simulink model "InsulinPumpModelV7_ParFor"  (R2022b)
settings: Solver=ode23t  StartTime=0.0  StopTime=12  MaxStep=0.001  RelTol=1e-5  EnableMultiTasking=on
undefined symbols (not defined in the file): const_Occl_Pct, DeliveryType, DiscIntNeverNeededParam, MagB, PauseTime, reserv_str, StrokeTimeB
libraries: fl_lib x71, nesl_utility x35, sldvlib x14, sh_lib x9, fl_ps_legacy_lib x8, sdl_lib x7, ee_lib x1, simulink_extras x1, simulink x1, slpidlib x1
(part 2 of 2)

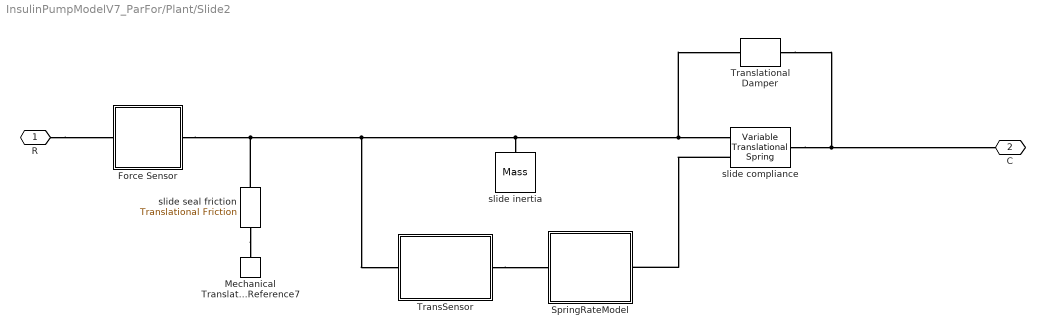
== system InsulinPumpModelV7_ParFor/Plant/Slide2 ==
  Force Sensor : Subsystem
  Mechanical Translational Reference7 : fl_lib/Mechanical/Translational Elements/Mechanical Translational Reference
  SpringRateModel : Subsystem  mask{E=reserv_str.Slide.EMod, A=reserv_str.Slide.CrosA, InitL=reserv_str.Slide.InitL}
      mask prompts: E "Young's Modulus (Pa)"; A "Cross-sectional Area (m^2)"; InitL "Initial Length (m)"
  TransSensor : Subsystem
  Translational Damper : sdl_lib/Couplings & Drives/Springs & Dampers/Translational Damper  D=10000 N/(m/s)  enable_faults=0  b_fault=1e6 N/(m/s)  temporal_fault=0  fault_time=5 s  shock_fault=0  acceleration_limit=100 m/s^2  shock_limit=1  report_fault=(1)-1  thermal_port=simscape.enum.thermaleffects.omit  thermal_mass=50 kJ/K  temperature_specify=off  temperature_priority=High  temperature=300 K  temperature_nominal_specify=off  temperature_nominal_unit=K  temperature_nominal_value=1
  slide compliance : sdl_lib/Couplings & Drives/Springs & Dampers/Variable Translational Spring  Kmin=reserv_str.Slide.MinSprRate N/m  x_specify=on  x_priority=High  x=reserv_str.Slide.InitDeform mm  x_nominal_specify=off  x_nominal_unit=m  x_nominal_value=1
      settings: InternalSimscapePortConfiguration="{\"Bottom\":[],\"Left\":[{\"id\":\"K\",\"label\":\"K\",\"type\":\"input\"},{\"id\":\"R\",\"label\":\"R\",\"type\":\"foundation.mechanical.translational.translational\"}],\"Right\":[{\"id\":\"C\",\"label\":\"C\",\"type\":\"foundation.mechanical.translational.translational\"}],\"Top\":[]}"
  slide inertia : fl_lib/Mechanical/Translational Elements/Mass  mass=reserv_str.Slide.Mass kg  num_ports=foundation.enum.numPorts2.one  v_specify=on  v_priority=High  v=0 m/s  v_nominal_specify=off  v_nominal_unit=m/s  v_nominal_value=1  f_specify=off  f_priority=High  f=0 N  f_nominal_specify=off  f_nominal_unit=N  f_nominal_value=1
  slide seal friction : fl_lib/Mechanical/Translational Elements/Translational Friction  brkwy_frc=reserv_str.Slide.Brkaway N  brkwy_vel=exp(-( (reserv_str.Slide.LinVelThresh) * 1 * (reserv_str.Slide.TransApproxCoeff) * 1 + 1/2) ) * ( (reserv_str.Slide.LinVelThresh) * 1 / 2 + 1 / ( (reserv_str.Slide.TransApproxCoeff) * 1) ) m/s  Col_frc=reserv_str.Slide.Coulomb N  visc_coef=reserv_str.Slide.ViscFric N/(m/s)  v_specify=off  v_priority=High  v=0 m/s  v_nominal_specify=off  v_nominal_unit=m/s  v_nominal_value=1  f_specify=off  f_priority=High  f=0 N  f_nominal_specify=off  f_nominal_unit=N  f_nominal_value=1
      settings: InternalSimscapePortConfiguration="{\"Bottom\":[],\"Left\":[{\"id\":\"R\",\"label\":\"R\",\"type\":\"foundation.mechanical.translational.translational\"}],\"Right\":[{\"id\":\"C\",\"label\":\"C\",\"type\":\"foundation.mechanical.translational.translational\"}],\"Top\":[]}"
  R : PMIOPort  Side=Left
  C : PMIOPort  Port=2  Side=Right
  connections:
  R/RConn1 -- Force Sensor/LConn1
  slide seal friction/RConn1 -- Mechanical Translational Reference7/LConn1
  TransSensor/RConn1 -- SpringRateModel/LConn1
  slide compliance/LConn1 -- SpringRateModel/RConn1
  Translational Damper/RConn1 -- C/RConn1 -- slide compliance/RConn1
  slide inertia/LConn1 -- slide compliance/LConn2 -- Translational Damper/LConn1 -- TransSensor/LConn1 -- slide seal friction/LConn1 -- Force Sensor/RConn1

== system InsulinPumpModelV7_ParFor/Plant/Slide3 ==
  Force Sensor : Subsystem
  Mechanical Translational Reference7 : fl_lib/Mechanical/Translational Elements/Mechanical Translational Reference
  SpringRateModel : Subsystem  mask{E=reserv_str.Slide.EMod, A=reserv_str.Slide.CrosA, InitL=reserv_str.Slide.InitL}
      mask prompts: E "Young's Modulus (Pa)"; A "Cross-sectional Area (m^2)"; InitL "Initial Length (m)"
  TransSensor : Subsystem
  Translational Damper : sdl_lib/Couplings & Drives/Springs & Dampers/Translational Damper  D=1 N/(m/s)  enable_faults=0  b_fault=1e6 N/(m/s)  temporal_fault=0  fault_time=5 s  shock_fault=0  acceleration_limit=100 m/s^2  shock_limit=1  report_fault=(1)-1  thermal_port=simscape.enum.thermaleffects.omit  thermal_mass=50 kJ/K  temperature_specify=off  temperature_priority=High  temperature=300 K  temperature_nominal_specify=off  temperature_nominal_unit=K  temperature_nominal_value=1
  slide compliance : sdl_lib/Couplings & Drives/Springs & Dampers/Variable Translational Spring  Kmin=reserv_str.Slide.MinSprRate N/m  x_specify=on  x_priority=High  x=reserv_str.Slide.InitDeform mm  x_nominal_specify=off  x_nominal_unit=m  x_nominal_value=1
      settings: InternalSimscapePortConfiguration="{\"Bottom\":[],\"Left\":[{\"id\":\"K\",\"label\":\"K\",\"type\":\"input\"},{\"id\":\"R\",\"label\":\"R\",\"type\":\"foundation.mechanical.translational.translational\"}],\"Right\":[{\"id\":\"C\",\"label\":\"C\",\"type\":\"foundation.mechanical.translational.translational\"}],\"Top\":[]}"
  slide inertia : fl_lib/Mechanical/Translational Elements/Mass  mass=reserv_str.Slide.Mass kg  num_ports=foundation.enum.numPorts2.one  v_specify=on  v_priority=High  v=0 m/s  v_nominal_specify=off  v_nominal_unit=m/s  v_nominal_value=1  f_specify=off  f_priority=High  f=0 N  f_nominal_specify=off  f_nominal_unit=N  f_nominal_value=1
  slide seal friction : fl_lib/Mechanical/Translational Elements/Translational Friction  brkwy_frc=reserv_str.Slide.Brkaway N  brkwy_vel=exp(-( (reserv_str.Slide.LinVelThresh) * 1 * (reserv_str.Slide.TransApproxCoeff) * 1 + 1/2) ) * ( (reserv_str.Slide.LinVelThresh) * 1 / 2 + 1 / ( (reserv_str.Slide.TransApproxCoeff) * 1) ) m/s  Col_frc=reserv_str.Slide.Coulomb N  visc_coef=reserv_str.Slide.ViscFric N/(m/s)  v_specify=off  v_priority=High  v=0 m/s  v_nominal_specify=off  v_nominal_unit=m/s  v_nominal_value=1  f_specify=off  f_priority=High  f=0 N  f_nominal_specify=off  f_nominal_unit=N  f_nominal_value=1
      settings: InternalSimscapePortConfiguration="{\"Bottom\":[],\"Left\":[{\"id\":\"R\",\"label\":\"R\",\"type\":\"foundation.mechanical.translational.translational\"}],\"Right\":[{\"id\":\"C\",\"label\":\"C\",\"type\":\"foundation.mechanical.translational.translational\"}],\"Top\":[]}"
  R : PMIOPort  Side=Left
  C : PMIOPort  Port=2  Side=Right
  connections:
  R/RConn1 -- Force Sensor/LConn1
  slide seal friction/RConn1 -- Mechanical Translational Reference7/LConn1
  TransSensor/RConn1 -- SpringRateModel/LConn1
  slide compliance/LConn1 -- SpringRateModel/RConn1
  Translational Damper/RConn1 -- C/RConn1 -- slide compliance/RConn1
  slide seal friction/LConn1 -- Translational Damper/LConn1 -- slide compliance/LConn2 -- slide inertia/LConn1 -- TransSensor/LConn1 -- Force Sensor/RConn1

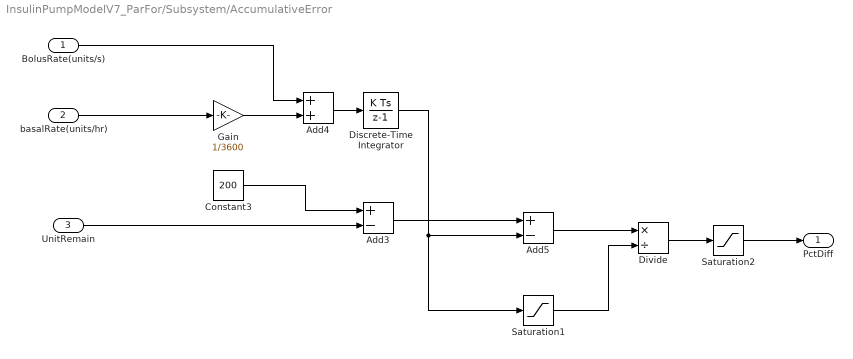
== system InsulinPumpModelV7_ParFor/Subsystem/AccumulativeError ==
  BolusRate(units/s) : Inport
  basalRate(units/hr) : Inport  Port=2
  UnitRemain : Inport  Port=3
  Add3 : Sum  Inputs=+-
  Add4 : Sum
  Add5 : Sum  Inputs=+-
  Constant3 : Constant  Value=200
  Discrete-Time Integrator : DiscreteIntegrator  SampleTime=-1  ICPrevOutput=DiscIntNeverNeededParam  ICPrevScaledInput=DiscIntNeverNeededParam
  Divide : Product  Inputs=*/
  Gain : Gain  Gain=1/3600
  Saturation1 : Saturate  UpperLimit=200  LowerLimit=0.000001
  Saturation2 : Saturate  UpperLimit=1  LowerLimit=-1
  PctDiff : Outport
  wires:
  Divide/1 -> Saturation2/1
  Saturation1/1 -> Divide/2
  UnitRemain/1 -> Add3/2
  basalRate(units/hr)/1 -> Gain/1
  BolusRate(units/s)/1 -> Add4/1
  Add4/1 -> Discrete-Time Integrator/1
  Discrete-Time Integrator/1 -> Add5/2, Saturation1/1
  Add3/1 -> Add5/1
  Constant3/1 -> Add3/1
  Saturation2/1 -> PctDiff/1
  Gain/1 -> Add4/2
  Add5/1 -> Divide/1

== system InsulinPumpModelV7_ParFor/Subsystem/Disp2Unit ==
  Piston_P : Inport  OutMin=-30  OutMax=0
  Add2 : Sum  Inputs=+-
  Add3 : Sum
  Constant : Constant  Value=reserv_str.Resvor.Vol  OutDataTypeStr=single
  Constant1 : Constant  Value=reserv_str.Resvor.Len  OutDataTypeStr=single
  Gain : Gain  Gain=reserv_str.Resvor.Area
  Gain1 : Gain  Gain=1/15
  Scope2 : Scope
  NumU : Outport  OutMin=0  OutMax=201
  wires:
  Constant/1 -> Add2/1
  Constant1/1 -> Add3/2
  Gain/1 -> Add2/2
  Add2/1 -> Gain1/1
  Gain1/1 -> NumU/1
  Add3/1 -> Gain/1, Scope2/1
  Piston_P/1 -> Add3/1

== system InsulinPumpModelV7_ParFor/Subsystem/SpeedController ==
  RefASpd : Inport  OutMin=-6000  OutMax=6000
  ASpd : Inport  Port=2  OutMin=-6000  OutMax=6000
  Add1 : Sum
  Discrete Transfer Fcn2 : DiscreteTransferFcn  Numerator=[0.367879441171442,0.264241117657115]  Denominator=[1,-0.367879441171442]  SampleTime=0.001
  FeedbackController : Subsystem
  Rate Limiter : RateLimiter  RisingSlewLimit=10  FallingSlewLimit=-10  SampleTimeMode=inherited
  Reference_motor_speed_limit : Saturate  UpperLimit=5200  LowerLimit=-5200
  SteadyStateLookup : Lookup_n-D  NumberOfTableDimensions=1  BreakpointsForDimension1=[0 0.136 0.170 0.205 1.08 2.58 8.02 12.8 33.8 828.2 1535.4 2171.5 2526 3000 3827.2 4246 4775.6 4991.1 5209.4]  Table=[0 0.25 0.3 0.35 0.355 0.36 0.38 0.4 0.5 1 1.5 2 2.3 2.72 3.5 3.9 4.4 4.6 4.8]  ExtrapMethod=Clip  InternalRulePriority=Speed  RndMeth=Simplest
  Volt : Outport  OutMin=-10  OutMax=10
  wires:
  RefASpd/1 -> Reference_motor_speed_limit/1
  SteadyStateLookup/1 -> Add1/1
  Discrete Transfer Fcn2/1 -> FeedbackController/1(RefASpd), SteadyStateLookup/1
  Add1/1 -> Rate Limiter/1
  Rate Limiter/1 -> Volt/1
  Reference_motor_speed_limit/1 -> Discrete Transfer Fcn2/1
  FeedbackController/1(Volt) -> Add1/2
  ASpd/1 -> FeedbackController/2(ASpd)

== system InsulinPumpModelV7_ParFor/Subsystem/Units_Conversion ==
  StokeMag : Inport  OutMin=0  OutMax=15
  BasalRate : Inport  Port=2  OutMin=0  OutMax=2
  Add2 : Sum
  BasalMap2Spd : Subsystem
  BolusMap2Spd : Subsystem
  RefASpd : Outport  OutMin=-6000  OutMax=6000
  wires:
  BasalMap2Spd/1(rev/min) -> Add2/2
  BolusMap2Spd/1(rev/min) -> Add2/1
  StokeMag/1 -> BolusMap2Spd/1(unit/s)
  BasalRate/1 -> BasalMap2Spd/1(unit/hr)
  Add2/1 -> RefASpd/1

== system InsulinPumpModelV7_ParFor/Plant/DC Motor Drive/AngSensor ==
  Ideal Rotational Motion Sensor : fl_lib/Mechanical/Mechanical Sensors/Ideal Rotational Motion Sensor  reference=foundation.enum.MeasurementReference.difference  acceleration_port=false  velocity_port=true  position_port=true  wrap_angle=false  offset=0 rad
  Mechanical Rotational Reference1 : fl_lib/Mechanical/Rotational Elements/Mechanical Rotational Reference
  PS-Simulink Converter1 : nesl_utility/PS-Simulink Converter  PhysicalDomain=network_engine_domain  SubClassName=ps_output  LeftPortType=input  RightPortType=output  PseudoPeriodic=off  Frequencies=[]  VectorFormat=1-D array  Unit=rad  AffineConversion=off
  PS-Simulink Converter9 : nesl_utility/PS-Simulink Converter  PhysicalDomain=network_engine_domain  SubClassName=ps_output  LeftPortType=input  RightPortType=output  PseudoPeriodic=off  Frequencies=[]  VectorFormat=1-D array  Unit=rpm  AffineConversion=off
  Terminator1 : Terminator
  R : PMIOPort  Side=Left
  ASpd : Outport
  wires:
  PS-Simulink Converter1/1 -> Terminator1/1  "DCMotor_APos"
  PS-Simulink Converter9/1 -> ASpd/1  "DCMotor_ASpd"
  connections:
  Mechanical Rotational Reference1/LConn1 -- Ideal Rotational Motion Sensor/RConn1
  Ideal Rotational Motion Sensor/RConn2 -- PS-Simulink Converter9/LConn1
  Ideal Rotational Motion Sensor/RConn3 -- PS-Simulink Converter1/LConn1
  R/RConn1 -- Ideal Rotational Motion Sensor/LConn1

== system InsulinPumpModelV7_ParFor/Plant/DC Motor Drive/CurrSensor ==
  Current Sensor1 : fl_lib/Electrical/Electrical Sensors/Current Sensor
  PS-Simulink Converter11 : nesl_utility/PS-Simulink Converter  PhysicalDomain=network_engine_domain  SubClassName=ps_output  LeftPortType=input  RightPortType=output  PseudoPeriodic=off  Frequencies=[]  VectorFormat=1-D array  Unit=A  AffineConversion=off
  Terminator : Terminator
  + : PMIOPort  Side=Left
  - : PMIOPort  Port=2  Side=Right
  wires:
  PS-Simulink Converter11/1 -> Terminator/1
  connections:
  Current Sensor1/RConn2 -- -/RConn1
  Current Sensor1/LConn1 -- +/RConn1
  Current Sensor1/RConn1 -- PS-Simulink Converter11/LConn1

== system InsulinPumpModelV7_ParFor/Plant/DC Motor Drive/TrqSensor ==
  Ideal Torque Sensor1 : fl_lib/Mechanical/Mechanical Sensors/Ideal Torque Sensor
  PS-Simulink Converter10 : nesl_utility/PS-Simulink Converter  PhysicalDomain=network_engine_domain  SubClassName=ps_output  LeftPortType=input  RightPortType=output  PseudoPeriodic=off  Frequencies=[]  VectorFormat=1-D array  Unit=N*m  AffineConversion=off
  Terminator : Terminator
  C : PMIOPort  Side=Right
  R : PMIOPort  Port=2  Side=Left
  wires:
  PS-Simulink Converter10/1 -> Terminator/1  "DCMotor_Torque"
  connections:
  Ideal Torque Sensor1/RConn1 -- C/RConn1
  Ideal Torque Sensor1/RConn2 -- PS-Simulink Converter10/LConn1
  Ideal Torque Sensor1/LConn1 -- R/RConn1

== system InsulinPumpModelV7_ParFor/Plant/DeliveryLine/FlowSensor#0 ==
  Hydraulic Flow Rate Sensor : fl_lib/Hydraulic/Hydraulic Sensors/Hydraulic Flow Rate Sensor
  PS-Simulink Converter : nesl_utility/PS-Simulink Converter  PhysicalDomain=network_engine_domain  SubClassName=ps_output  LeftPortType=input  RightPortType=output  PseudoPeriodic=off  Frequencies=[]  VectorFormat=1-D array  Unit=mm^3/min  AffineConversion=off
  Saturation : Saturate  UpperLimit=inf  LowerLimit=0
  Scope : Scope
  A : PMIOPort  Side=Left
  B : PMIOPort  Port=2  Side=Right
  wires:
  PS-Simulink Converter/1 -> Saturation/1
  Saturation/1 -> Scope/1
  connections:
  Hydraulic Flow Rate Sensor/RConn1 -- PS-Simulink Converter/LConn1
  Hydraulic Flow Rate Sensor/RConn2 -- B/RConn1
  A/RConn1 -- Hydraulic Flow Rate Sensor/LConn1

== system InsulinPumpModelV7_ParFor/Plant/DeliveryLine/FlowSensor#1 ==
  Hydraulic Flow Rate Sensor : fl_lib/Hydraulic/Hydraulic Sensors/Hydraulic Flow Rate Sensor
  PS-Simulink Converter : nesl_utility/PS-Simulink Converter  PhysicalDomain=network_engine_domain  SubClassName=ps_output  LeftPortType=input  RightPortType=output  PseudoPeriodic=off  Frequencies=[]  VectorFormat=1-D array  Unit=mm^3/min  AffineConversion=off
  Saturation : Saturate  Commented=through  UpperLimit=5000  LowerLimit=0
  Scope : Scope
  A : PMIOPort  Side=Left
  B : PMIOPort  Port=2  Side=Right
  wires:
  PS-Simulink Converter/1 -> Saturation/1
  Saturation/1 -> Scope/1
  connections:
  A/RConn1 -- Hydraulic Flow Rate Sensor/LConn1
  Hydraulic Flow Rate Sensor/RConn2 -- B/RConn1
  Hydraulic Flow Rate Sensor/RConn1 -- PS-Simulink Converter/LConn1

== system InsulinPumpModelV7_ParFor/Plant/DeliveryLine/P Sensor ==
  Hydraulic Pressure Sensor : fl_lib/Hydraulic/Hydraulic Sensors/Hydraulic Pressure Sensor
  Hydraulic Reference : fl_lib/Hydraulic/Hydraulic Elements/Hydraulic Reference
  PS-Simulink Converter : nesl_utility/PS-Simulink Converter  PhysicalDomain=network_engine_domain  SubClassName=ps_output  LeftPortType=input  RightPortType=output  PseudoPeriodic=off  Frequencies=[]  VectorFormat=1-D array  Unit=1  AffineConversion=off
  A : PMIOPort  Side=Left
  P : Outport
  wires:
  PS-Simulink Converter/1 -> P/1  "Press2"
  connections:
  Hydraulic Pressure Sensor/RConn1 -- Hydraulic Reference/LConn1
  Hydraulic Pressure Sensor/RConn2 -- PS-Simulink Converter/LConn1
  A/RConn1 -- Hydraulic Pressure Sensor/LConn1

== system InsulinPumpModelV7_ParFor/Plant/Drive System/AngSensor ==
  Ideal Rotational Motion Sensor : fl_lib/Mechanical/Mechanical Sensors/Ideal Rotational Motion Sensor  reference=foundation.enum.MeasurementReference.difference  acceleration_port=false  velocity_port=true  position_port=true  wrap_angle=false  offset=0 rad
  Mechanical Rotational Reference1 : fl_lib/Mechanical/Rotational Elements/Mechanical Rotational Reference
  PS-Simulink Converter1 : nesl_utility/PS-Simulink Converter  PhysicalDomain=network_engine_domain  SubClassName=ps_output  LeftPortType=input  RightPortType=output  PseudoPeriodic=off  Frequencies=[]  VectorFormat=1-D array  Unit=rad  AffineConversion=off
  PS-Simulink Converter9 : nesl_utility/PS-Simulink Converter  PhysicalDomain=network_engine_domain  SubClassName=ps_output  LeftPortType=input  RightPortType=output  PseudoPeriodic=off  Frequencies=[]  VectorFormat=1-D array  Unit=rpm  AffineConversion=off
  Scope : Scope
  Scope1 : Scope
  Terminator : Terminator
  Terminator1 : Terminator
  Conn1 : PMIOPort  Side=Left
  wires:
  PS-Simulink Converter1/1 -> Scope1/1, Terminator1/1  "Inertia_APos"
  PS-Simulink Converter9/1 -> Scope/1, Terminator/1  "Inertia_ASpd"
  connections:
  Mechanical Rotational Reference1/LConn1 -- Ideal Rotational Motion Sensor/RConn1
  Ideal Rotational Motion Sensor/RConn2 -- PS-Simulink Converter9/LConn1
  Ideal Rotational Motion Sensor/RConn3 -- PS-Simulink Converter1/LConn1
  Conn1/RConn1 -- Ideal Rotational Motion Sensor/LConn1

== system InsulinPumpModelV7_ParFor/Plant/Reservoir1/P Sensor ==
  Hydraulic Pressure Sensor : fl_lib/Hydraulic/Hydraulic Sensors/Hydraulic Pressure Sensor
  Hydraulic Reference : fl_lib/Hydraulic/Hydraulic Elements/Hydraulic Reference
  PS-Simulink Converter : nesl_utility/PS-Simulink Converter  PhysicalDomain=network_engine_domain  SubClassName=ps_output  LeftPortType=input  RightPortType=output  PseudoPeriodic=off  Frequencies=[]  VectorFormat=1-D array  Unit=1  AffineConversion=off
  Scope1 : Scope
  A : PMIOPort  Side=Left
  wires:
  PS-Simulink Converter/1 -> Scope1/1  "Press1"
  connections:
  Hydraulic Pressure Sensor/RConn1 -- Hydraulic Reference/LConn1
  Hydraulic Pressure Sensor/RConn2 -- PS-Simulink Converter/LConn1
  A/RConn1 -- Hydraulic Pressure Sensor/LConn1

== system InsulinPumpModelV7_ParFor/Plant/Reservoir1/TransSensor ==
  Ideal Translational Motion Sensor : fl_lib/Mechanical/Mechanical Sensors/Ideal Translational Motion Sensor  reference=foundation.enum.MeasurementReference.difference  acceleration_port=false  velocity_port=true  position_port=true  offset=0 m
  Mechanical Translational Reference1 : fl_lib/Mechanical/Translational Elements/Mechanical Translational Reference
  PS-Simulink Converter3 : nesl_utility/PS-Simulink Converter  PhysicalDomain=network_engine_domain  SubClassName=ps_output  LeftPortType=input  RightPortType=output  PseudoPeriodic=off  Frequencies=[]  VectorFormat=1-D array  Unit=mm/min  AffineConversion=off
  PS-Simulink Converter4 : nesl_utility/PS-Simulink Converter  PhysicalDomain=network_engine_domain  SubClassName=ps_output  LeftPortType=input  RightPortType=output  PseudoPeriodic=off  Frequencies=[]  VectorFormat=1-D array  Unit=mm  AffineConversion=off
  Scope : Scope
  Scope1 : Scope
  Terminator : Terminator
  Terminator1 : Terminator
  Conn1 : PMIOPort  Side=Left
  P : PMIOPort  Port=2  Side=Right
  wires:
  PS-Simulink Converter4/1 -> Scope1/1, Terminator1/1  "Piston_P"
  PS-Simulink Converter3/1 -> Scope/1, Terminator/1  "Piston_V"
  connections:
  Conn1/RConn1 -- Ideal Translational Motion Sensor/LConn1
  Ideal Translational Motion Sensor/RConn3 -- P/RConn1 -- PS-Simulink Converter4/LConn1
  PS-Simulink Converter3/LConn1 -- Ideal Translational Motion Sensor/RConn2
  Mechanical Translational Reference1/LConn1 -- Ideal Translational Motion Sensor/RConn1

== system InsulinPumpModelV7_ParFor/Plant/Reservoir2/P Sensor ==
  Hydraulic Pressure Sensor : fl_lib/Hydraulic/Hydraulic Sensors/Hydraulic Pressure Sensor
  Hydraulic Reference : fl_lib/Hydraulic/Hydraulic Elements/Hydraulic Reference
  PS-Simulink Converter : nesl_utility/PS-Simulink Converter  PhysicalDomain=network_engine_domain  SubClassName=ps_output  LeftPortType=input  RightPortType=output  PseudoPeriodic=off  Frequencies=[]  VectorFormat=1-D array  Unit=1  AffineConversion=off
  Scope1 : Scope
  A : PMIOPort  Side=Left
  wires:
  PS-Simulink Converter/1 -> Scope1/1  "Press1"
  connections:
  A/RConn1 -- Hydraulic Pressure Sensor/LConn1
  Hydraulic Pressure Sensor/RConn2 -- PS-Simulink Converter/LConn1
  Hydraulic Pressure Sensor/RConn1 -- Hydraulic Reference/LConn1

== system InsulinPumpModelV7_ParFor/Plant/Reservoir2/TransSensor ==
  Ideal Translational Motion Sensor : fl_lib/Mechanical/Mechanical Sensors/Ideal Translational Motion Sensor  reference=foundation.enum.MeasurementReference.difference  acceleration_port=false  velocity_port=true  position_port=true  offset=0 m
  Mechanical Translational Reference1 : fl_lib/Mechanical/Translational Elements/Mechanical Translational Reference
  PS-Simulink Converter3 : nesl_utility/PS-Simulink Converter  PhysicalDomain=network_engine_domain  SubClassName=ps_output  LeftPortType=input  RightPortType=output  PseudoPeriodic=off  Frequencies=[]  VectorFormat=1-D array  Unit=mm/min  AffineConversion=off
  PS-Simulink Converter4 : nesl_utility/PS-Simulink Converter  PhysicalDomain=network_engine_domain  SubClassName=ps_output  LeftPortType=input  RightPortType=output  PseudoPeriodic=off  Frequencies=[]  VectorFormat=1-D array  Unit=mm  AffineConversion=off
  Scope : Scope
  Scope1 : Scope
  Terminator : Terminator
  Terminator1 : Terminator
  Conn1 : PMIOPort  Side=Left
  P : PMIOPort  Port=2  Side=Right
  wires:
  PS-Simulink Converter3/1 -> Terminator/1, Scope/1  "Piston_V"
  PS-Simulink Converter4/1 -> Terminator1/1, Scope1/1  "Piston_P"
  connections:
  Mechanical Translational Reference1/LConn1 -- Ideal Translational Motion Sensor/RConn1
  PS-Simulink Converter3/LConn1 -- Ideal Translational Motion Sensor/RConn2
  PS-Simulink Converter4/LConn1 -- P/RConn1 -- Ideal Translational Motion Sensor/RConn3
  Conn1/RConn1 -- Ideal Translational Motion Sensor/LConn1

== system InsulinPumpModelV7_ParFor/Plant/Reservoir3/P Sensor ==
  Hydraulic Pressure Sensor : fl_lib/Hydraulic/Hydraulic Sensors/Hydraulic Pressure Sensor
  Hydraulic Reference : fl_lib/Hydraulic/Hydraulic Elements/Hydraulic Reference
  PS-Simulink Converter : nesl_utility/PS-Simulink Converter  PhysicalDomain=network_engine_domain  SubClassName=ps_output  LeftPortType=input  RightPortType=output  PseudoPeriodic=off  Frequencies=[]  VectorFormat=1-D array  Unit=1  AffineConversion=off
  Scope1 : Scope
  A : PMIOPort  Side=Left
  wires:
  PS-Simulink Converter/1 -> Scope1/1  "Press1"
  connections:
  A/RConn1 -- Hydraulic Pressure Sensor/LConn1
  Hydraulic Pressure Sensor/RConn2 -- PS-Simulink Converter/LConn1
  Hydraulic Pressure Sensor/RConn1 -- Hydraulic Reference/LConn1

== system InsulinPumpModelV7_ParFor/Plant/Reservoir3/TransSensor ==
  Ideal Translational Motion Sensor : fl_lib/Mechanical/Mechanical Sensors/Ideal Translational Motion Sensor  reference=foundation.enum.MeasurementReference.difference  acceleration_port=false  velocity_port=true  position_port=true  offset=0 m
  Mechanical Translational Reference1 : fl_lib/Mechanical/Translational Elements/Mechanical Translational Reference
  PS-Simulink Converter3 : nesl_utility/PS-Simulink Converter  PhysicalDomain=network_engine_domain  SubClassName=ps_output  LeftPortType=input  RightPortType=output  PseudoPeriodic=off  Frequencies=[]  VectorFormat=1-D array  Unit=mm/min  AffineConversion=off
  PS-Simulink Converter4 : nesl_utility/PS-Simulink Converter  PhysicalDomain=network_engine_domain  SubClassName=ps_output  LeftPortType=input  RightPortType=output  PseudoPeriodic=off  Frequencies=[]  VectorFormat=1-D array  Unit=mm  AffineConversion=off
  Scope : Scope
  Scope1 : Scope
  Terminator : Terminator
  Terminator1 : Terminator
  Conn1 : PMIOPort  Side=Left
  P : PMIOPort  Port=2  Side=Right
  wires:
  PS-Simulink Converter3/1 -> Terminator/1, Scope/1  "Piston_V"
  PS-Simulink Converter4/1 -> Terminator1/1, Scope1/1  "Piston_P"
  connections:
  Mechanical Translational Reference1/LConn1 -- Ideal Translational Motion Sensor/RConn1
  PS-Simulink Converter3/LConn1 -- Ideal Translational Motion Sensor/RConn2
  PS-Simulink Converter4/LConn1 -- P/RConn1 -- Ideal Translational Motion Sensor/RConn3
  Conn1/RConn1 -- Ideal Translational Motion Sensor/LConn1

== system InsulinPumpModelV7_ParFor/Plant/Slide1/Force Sensor ==
  Ideal Force Sensor1 : fl_lib/Mechanical/Mechanical Sensors/Ideal Force Sensor
  PS-Simulink Converter15 : nesl_utility/PS-Simulink Converter  PhysicalDomain=network_engine_domain  SubClassName=ps_output  LeftPortType=input  RightPortType=output  PseudoPeriodic=off  Frequencies=[]  VectorFormat=1-D array  Unit=N  AffineConversion=off
  Rate Transition4 : RateTransition  OutPortSampleTime=0.01
  Scope2 : Scope
  Terminator : Terminator
  C : PMIOPort  Side=Right
  R : PMIOPort  Port=2  Side=Left
  wires:
  PS-Simulink Converter15/1 -> Rate Transition4/1, Terminator/1  "Slide_Force"
  Rate Transition4/1 -> Scope2/1
  connections:
  Ideal Force Sensor1/LConn1 -- R/RConn1
  PS-Simulink Converter15/LConn1 -- Ideal Force Sensor1/RConn2
  C/RConn1 -- Ideal Force Sensor1/RConn1

== system InsulinPumpModelV7_ParFor/Plant/Slide2/Force Sensor ==
  Ideal Force Sensor1 : fl_lib/Mechanical/Mechanical Sensors/Ideal Force Sensor
  PS-Simulink Converter15 : nesl_utility/PS-Simulink Converter  PhysicalDomain=network_engine_domain  SubClassName=ps_output  LeftPortType=input  RightPortType=output  PseudoPeriodic=off  Frequencies=[]  VectorFormat=1-D array  Unit=N  AffineConversion=off
  Rate Transition4 : RateTransition  OutPortSampleTime=0.01
  Scope2 : Scope
  Terminator : Terminator
  C : PMIOPort  Side=Right
  R : PMIOPort  Port=2  Side=Left
  wires:
  Rate Transition4/1 -> Scope2/1
  PS-Simulink Converter15/1 -> Terminator/1, Rate Transition4/1  "Slide_Force"
  connections:
  C/RConn1 -- Ideal Force Sensor1/RConn1
  PS-Simulink Converter15/LConn1 -- Ideal Force Sensor1/RConn2
  Ideal Force Sensor1/LConn1 -- R/RConn1

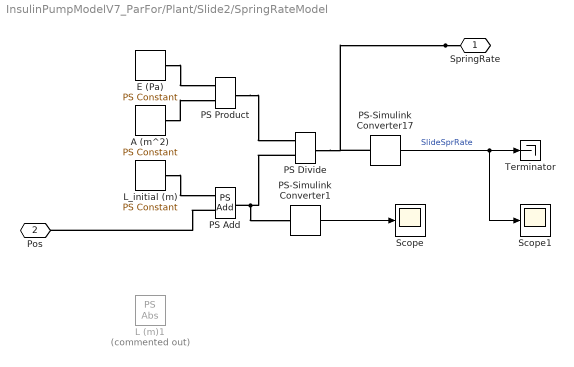
== system InsulinPumpModelV7_ParFor/Plant/Slide2/SpringRateModel ==
  A (m^2) : fl_lib/Physical Signals/Sources/PS Constant  constant=A
  E (Pa) : fl_lib/Physical Signals/Sources/PS Constant  constant=E
  L (m)1 : fl_ps_legacy_lib/Legacy Physical Signals/Nonlinear Operators/PS Abs  Commented=on
      settings: InternalSimscapePortConfiguration="{\"Bottom\":[],\"Left\":[{\"id\":\"I\",\"label\":\"\",\"type\":\"input\"}],\"Right\":[{\"id\":\"O\",\"label\":\"\",\"type\":\"output\"}],\"Top\":[]}"
  L_initial (m) : fl_lib/Physical Signals/Sources/PS Constant  constant=InitL
  PS Add : fl_ps_legacy_lib/Legacy Physical Signals/Functions/PS Add
      settings: InternalSimscapePortConfiguration="{\"Bottom\":[],\"Left\":[{\"id\":\"I1\",\"label\":\"\",\"type\":\"input\"},{\"id\":\"I2\",\"label\":\"\",\"type\":\"input\"}],\"Right\":[{\"id\":\"O\",\"label\":\"\",\"type\":\"output\"}],\"Top\":[]}"
  PS Divide : fl_ps_legacy_lib/Legacy Physical Signals/Functions/PS Divide
      settings: InternalSimscapePortConfiguration="{\"Bottom\":[],\"Left\":[{\"id\":\"I1\",\"label\":\"\",\"type\":\"input\"},{\"id\":\"I2\",\"label\":\"\",\"type\":\"input\"}],\"Right\":[{\"id\":\"O\",\"label\":\"\",\"type\":\"output\"}],\"Top\":[]}"
  PS Product : fl_ps_legacy_lib/Legacy Physical Signals/Functions/PS Product
  PS-Simulink Converter1 : nesl_utility/PS-Simulink Converter  PhysicalDomain=network_engine_domain  SubClassName=ps_output  LeftPortType=input  RightPortType=output  PseudoPeriodic=off  Frequencies=[]  VectorFormat=1-D array  Unit=N/m  AffineConversion=off
  PS-Simulink Converter17 : nesl_utility/PS-Simulink Converter  PhysicalDomain=network_engine_domain  SubClassName=ps_output  LeftPortType=input  RightPortType=output  PseudoPeriodic=off  Frequencies=[]  VectorFormat=1-D array  Unit=N/m  AffineConversion=off
  Scope : Scope
  Scope1 : Scope
  Terminator : Terminator
  SpringRate : PMIOPort  Side=Right
  Pos : PMIOPort  Port=2  Side=Left
  wires:
  PS-Simulink Converter1/1 -> Scope/1
  PS-Simulink Converter17/1 -> Terminator/1, Scope1/1  "SlideSprRate"
  connections:
  PS Add/LConn2 -- Pos/RConn1
  PS Add/RConn1 -- PS-Simulink Converter1/LConn1 -- PS Divide/LConn2
  L_initial (m)/RConn1 -- PS Add/LConn1
  SpringRate/RConn1 -- PS-Simulink Converter17/LConn1 -- PS Divide/RConn1
  PS Product/RConn1 -- PS Divide/LConn1
  A (m^2)/RConn1 -- PS Product/LConn2
  E (Pa)/RConn1 -- PS Product/LConn1

== system InsulinPumpModelV7_ParFor/Plant/Slide2/TransSensor ==
  Ideal Translational Motion Sensor : fl_lib/Mechanical/Mechanical Sensors/Ideal Translational Motion Sensor  reference=foundation.enum.MeasurementReference.difference  acceleration_port=false  velocity_port=true  position_port=true  offset=0 m
  Mechanical Translational Reference1 : fl_lib/Mechanical/Translational Elements/Mechanical Translational Reference
  PS-Simulink Converter3 : nesl_utility/PS-Simulink Converter  PhysicalDomain=network_engine_domain  SubClassName=ps_output  LeftPortType=input  RightPortType=output  PseudoPeriodic=off  Frequencies=[]  VectorFormat=1-D array  Unit=mm/s  AffineConversion=off
  PS-Simulink Converter4 : nesl_utility/PS-Simulink Converter  PhysicalDomain=network_engine_domain  SubClassName=ps_output  LeftPortType=input  RightPortType=output  PseudoPeriodic=off  Frequencies=[]  VectorFormat=1-D array  Unit=mm  AffineConversion=off
  Terminator : Terminator
  Terminator1 : Terminator
  Conn1 : PMIOPort  Side=Left
  P : PMIOPort  Port=2  Side=Right
  wires:
  PS-Simulink Converter3/1 -> Terminator/1  "Slide_V"
  PS-Simulink Converter4/1 -> Terminator1/1  "Slide_P"
  connections:
  Mechanical Translational Reference1/LConn1 -- Ideal Translational Motion Sensor/RConn1
  PS-Simulink Converter3/LConn1 -- Ideal Translational Motion Sensor/RConn2
  PS-Simulink Converter4/LConn1 -- P/RConn1 -- Ideal Translational Motion Sensor/RConn3
  Conn1/RConn1 -- Ideal Translational Motion Sensor/LConn1

== system InsulinPumpModelV7_ParFor/Plant/Slide3/Force Sensor ==
  Ideal Force Sensor1 : fl_lib/Mechanical/Mechanical Sensors/Ideal Force Sensor
  PS-Simulink Converter15 : nesl_utility/PS-Simulink Converter  PhysicalDomain=network_engine_domain  SubClassName=ps_output  LeftPortType=input  RightPortType=output  PseudoPeriodic=off  Frequencies=[]  VectorFormat=1-D array  Unit=N  AffineConversion=off
  Rate Transition4 : RateTransition  OutPortSampleTime=0.01
  Scope2 : Scope
  Terminator : Terminator
  C : PMIOPort  Side=Right
  R : PMIOPort  Port=2  Side=Left
  wires:
  Rate Transition4/1 -> Scope2/1
  PS-Simulink Converter15/1 -> Terminator/1, Rate Transition4/1  "Slide_Force"
  connections:
  C/RConn1 -- Ideal Force Sensor1/RConn1
  PS-Simulink Converter15/LConn1 -- Ideal Force Sensor1/RConn2
  Ideal Force Sensor1/LConn1 -- R/RConn1

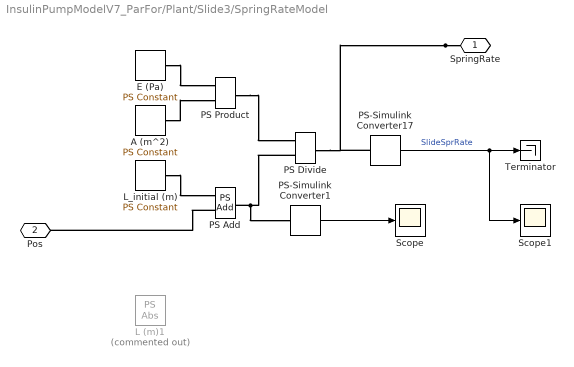
== system InsulinPumpModelV7_ParFor/Plant/Slide3/SpringRateModel ==
  A (m^2) : fl_lib/Physical Signals/Sources/PS Constant  constant=A
  E (Pa) : fl_lib/Physical Signals/Sources/PS Constant  constant=E
  L (m)1 : fl_ps_legacy_lib/Legacy Physical Signals/Nonlinear Operators/PS Abs  Commented=on
      settings: InternalSimscapePortConfiguration="{\"Bottom\":[],\"Left\":[{\"id\":\"I\",\"label\":\"\",\"type\":\"input\"}],\"Right\":[{\"id\":\"O\",\"label\":\"\",\"type\":\"output\"}],\"Top\":[]}"
  L_initial (m) : fl_lib/Physical Signals/Sources/PS Constant  constant=InitL
  PS Add : fl_ps_legacy_lib/Legacy Physical Signals/Functions/PS Add
      settings: InternalSimscapePortConfiguration="{\"Bottom\":[],\"Left\":[{\"id\":\"I1\",\"label\":\"\",\"type\":\"input\"},{\"id\":\"I2\",\"label\":\"\",\"type\":\"input\"}],\"Right\":[{\"id\":\"O\",\"label\":\"\",\"type\":\"output\"}],\"Top\":[]}"
  PS Divide : fl_ps_legacy_lib/Legacy Physical Signals/Functions/PS Divide
      settings: InternalSimscapePortConfiguration="{\"Bottom\":[],\"Left\":[{\"id\":\"I1\",\"label\":\"\",\"type\":\"input\"},{\"id\":\"I2\",\"label\":\"\",\"type\":\"input\"}],\"Right\":[{\"id\":\"O\",\"label\":\"\",\"type\":\"output\"}],\"Top\":[]}"
  PS Product : fl_ps_legacy_lib/Legacy Physical Signals/Functions/PS Product
  PS-Simulink Converter1 : nesl_utility/PS-Simulink Converter  PhysicalDomain=network_engine_domain  SubClassName=ps_output  LeftPortType=input  RightPortType=output  PseudoPeriodic=off  Frequencies=[]  VectorFormat=1-D array  Unit=N/m  AffineConversion=off
  PS-Simulink Converter17 : nesl_utility/PS-Simulink Converter  PhysicalDomain=network_engine_domain  SubClassName=ps_output  LeftPortType=input  RightPortType=output  PseudoPeriodic=off  Frequencies=[]  VectorFormat=1-D array  Unit=N/m  AffineConversion=off
  Scope : Scope
  Scope1 : Scope
  Terminator : Terminator
  SpringRate : PMIOPort  Side=Right
  Pos : PMIOPort  Port=2  Side=Left
  wires:
  PS-Simulink Converter1/1 -> Scope/1
  PS-Simulink Converter17/1 -> Terminator/1, Scope1/1  "SlideSprRate"
  connections:
  PS Add/LConn2 -- Pos/RConn1
  PS Add/RConn1 -- PS-Simulink Converter1/LConn1 -- PS Divide/LConn2
  L_initial (m)/RConn1 -- PS Add/LConn1
  SpringRate/RConn1 -- PS-Simulink Converter17/LConn1 -- PS Divide/RConn1
  PS Product/RConn1 -- PS Divide/LConn1
  A (m^2)/RConn1 -- PS Product/LConn2
  E (Pa)/RConn1 -- PS Product/LConn1

== system InsulinPumpModelV7_ParFor/Plant/Slide3/TransSensor ==
  Ideal Translational Motion Sensor : fl_lib/Mechanical/Mechanical Sensors/Ideal Translational Motion Sensor  reference=foundation.enum.MeasurementReference.difference  acceleration_port=false  velocity_port=true  position_port=true  offset=0 m
  Mechanical Translational Reference1 : fl_lib/Mechanical/Translational Elements/Mechanical Translational Reference
  PS-Simulink Converter3 : nesl_utility/PS-Simulink Converter  PhysicalDomain=network_engine_domain  SubClassName=ps_output  LeftPortType=input  RightPortType=output  PseudoPeriodic=off  Frequencies=[]  VectorFormat=1-D array  Unit=mm/s  AffineConversion=off
  PS-Simulink Converter4 : nesl_utility/PS-Simulink Converter  PhysicalDomain=network_engine_domain  SubClassName=ps_output  LeftPortType=input  RightPortType=output  PseudoPeriodic=off  Frequencies=[]  VectorFormat=1-D array  Unit=mm  AffineConversion=off
  Terminator : Terminator
  Terminator1 : Terminator
  Conn1 : PMIOPort  Side=Left
  P : PMIOPort  Port=2  Side=Right
  wires:
  PS-Simulink Converter3/1 -> Terminator/1  "Slide_V"
  PS-Simulink Converter4/1 -> Terminator1/1  "Slide_P"
  connections:
  Mechanical Translational Reference1/LConn1 -- Ideal Translational Motion Sensor/RConn1
  PS-Simulink Converter3/LConn1 -- Ideal Translational Motion Sensor/RConn2
  PS-Simulink Converter4/LConn1 -- P/RConn1 -- Ideal Translational Motion Sensor/RConn3
  Conn1/RConn1 -- Ideal Translational Motion Sensor/LConn1

== system InsulinPumpModelV7_ParFor/Subsystem/SpeedController/FeedbackController ==
  RefASpd : Inport  OutMin=-6000  OutMax=6000
  ASpd : Inport  Port=2  OutMin=-6000  OutMax=6000
  1-D Lookup Table : Lookup_n-D  NumberOfTableDimensions=1  BreakpointsForDimension1=[0 12.8 33.8 450]  Table=[1 1 1 1]*5e-4  InternalRulePriority=Speed  RndMeth=Simplest
  1-D Lookup Table1 : Lookup_n-D  NumberOfTableDimensions=1  BreakpointsForDimension1=[0 12.8 33.8 450]  Table=[1 1 1 1]*5e-4  InternalRulePriority=Speed  RndMeth=Simplest
  Add : Sum  Inputs=+-
  PID Controller : slpidlib/PID Controller  Controller=PI  Form=Parallel  TimeDomain=Discrete-time  UseExternalTs=off  SampleTime=0.001  IntegratorMethod=Forward Euler  FilterMethod=Forward Euler  ControllerParametersSource=external  P=2e-3  I=2e-3  UseKiTs=off  D=0  N=100  UseFilter=on  TunerSelectOption=Transfer Function Based (PID Tuner App)  InitialConditionSource=internal  InitialConditionForIntegrator=0  InitialConditionForFilter=0  DifferentiatorICPrevScaledInput=0  ExternalReset=none  TrackingMode=off  Kt=1  LimitOutput=off  SatLimitsSource=internal  UpperSaturationLimit=1  LowerSaturationLimit=1  LinearizeAsGain=on  AntiWindupMode=clamping  Kb=1  LimitIntegrator=off  UpperIntegratorSaturationLimit=inf  LowerIntegratorSaturationLimit=-inf  POutMin=[]  POutMax=[]  IOutMin=[]  IOutMax=[]  DOutMin=[]  DOutMax=[]  NOutMin=[]  NOutMax=[]  SumOutMin=[]  SumOutMax=[]  SaturationOutMin=[]  SaturationOutMax=[]  PParamMin=[]  PParamMax=[]  IParamMin=[]  IParamMax=[]  DParamMin=[]  DParamMax=[]  NParamMin=[]  NParamMax=[]  KbParamMin=[]  KbParamMax=[]  KtParamMin=[]  KtParamMax=[]  KbOutMin=[]  KbOutMax=[]  KtOutMin=[]  KtOutMax=[]  IntegratorOutMin=[]  IntegratorOutMax=[]  FilterOutMin=[]  FilterOutMax=[]  SumI1OutMin=[]  SumI1OutMax=[]  SumI2OutMin=[]  SumI2OutMax=[]  SumI3OutMin=[]  SumI3OutMax=[]  SumI4OutMin=[]  SumI4OutMax=[]  SumDOutMin=[]  SumDOutMax=[]  DifferentiatorOutMin=[]  DifferentiatorOutMax=[]  FilterDiffOutCoefMin=[]  FilterDiffOutCoefMax=[]  ReciprocalOutMin=[]  ReciprocalOutMax=[]  SumDenOutMin=[]  SumDenOutMax=[]  SumNumOutMin=[]  SumNumOutMax=[]  DivideOutMin=[]  DivideOutMax=[]  UdiffTsProdOutMin=[]  UdiffTsProdOutMax=[]  NTsProdOutMin=[]  NTsProdOutMax=[]  UintegralTsProdOutMin=[]  UintegralTsProdOutMax=[]  UngainTsProdOutMin=[]  UngainTsProdOutMax=[]  ClampingZeroOutDataTypeStr=Inherit: Inherit via back propagation  ClampingZeroOutMin=[]  ClampingZeroOutMax=[]  FilterDenConstantOutDataTypeStr=Inherit: Inherit via back propagation  FilterDenConstantOutMin=[]  FilterDenConstantOutMax=[]  PCopyOutDataTypeStr=Inherit: Inherit via back propagation  PCopyOutMin=[]  PCopyOutMax=[]  NCopyOutDataTypeStr=Inherit: Inherit via back propagation  NCopyOutMin=[]  NCopyOutMax=[]  IntegratorContinuousStateAttributes=''  IntegratorStateMustResolveToSignalObject=off  IntegratorRTWStateStorageClass=Auto  FilterContinuousStateAttributes=''  FilterStateMustResolveToSignalObject=off  FilterRTWStateStorageClass=Auto  ParallelPVariant=ExternalParameters  IdealPVariant=Disabled  IVariant=ExternalParameters  DVariant=Disabled  IntegratorVariant=Discrete  SatVariant=Disabled  AWVariant=Passthrough  PCopyVariant=Disabled  TRVariant=Disabled  FdbkBlocksVariant=Forward  IdealPFdbkVariant=Disabled  SatFdbkVariant=Disabled  DerivativeFilterVariant=Disabled  NVariant=Disabled  NCopyVariant=Disabled_SignalSpec  FilterICVariant=Disabled  IntegratorICVariant=InternalICs  ExternalResetVariant=Disabled  TRSumVariant=Passthrough  SumFdbkVariant=Disabled  SumVariant=Sum_PI  TsampFilterVariant=InternalTs  TsampNgainVariant=Passthrough  TsampIntegralVariant=Passthrough  ExternalSaturationOutDataTypeStr=Inherit: Same as second input
  Volt : Outport  OutMin=-10  OutMax=10
  wires:
  ASpd/1 -> Add/2
  Add/1 -> 1-D Lookup Table1/1, 1-D Lookup Table/1, PID Controller/1
  PID Controller/1 -> Volt/1
  1-D Lookup Table/1 -> PID Controller/2
  1-D Lookup Table1/1 -> PID Controller/3
  RefASpd/1 -> Add/1

== system InsulinPumpModelV7_ParFor/Subsystem/Units_Conversion/BasalMap2Spd ==
  unit/hr : Inport
  1/CrossArea_Output(mm/min) : Gain  Gain=1/reserv_str.Resvor.Area
  Gain : Gain  Gain=1/60
  Gain3 : Gain  Gain=15
  Gear_Input(rev/min) : Gain  Gain=reserv_str.DriveSys.GearRatio
  Rev/inch_Output(rev/min) : Gain  Gain=1/reserv_str.DriveSys.ScrewLead
  mm2inch_Output(inch/min) : Gain  Gain=1/25.4
  rev/min : Outport
  wires:
  Gain/1 -> Gain3/1
  Gain3/1 -> 1/CrossArea_Output(mm/min)/1  "mm^3/min"
  mm2inch_Output(inch/min)/1 -> Rev/inch_Output(rev/min)/1
  unit/hr/1 -> Gain/1
  1/CrossArea_Output(mm/min)/1 -> mm2inch_Output(inch/min)/1
  Rev/inch_Output(rev/min)/1 -> Gear_Input(rev/min)/1
  Gear_Input(rev/min)/1 -> rev/min/1

== system InsulinPumpModelV7_ParFor/Subsystem/Units_Conversion/BolusMap2Spd ==
  unit/s : Inport
  1/CrossArea_Output(mm/min) : Gain  Gain=1/reserv_str.Resvor.Area
  Gain : Gain  Gain=60
  Gain3 : Gain  Gain=15
  Gear_Input(rev/min) : Gain  Gain=reserv_str.DriveSys.GearRatio
  Rev/inch_Output(rev/min) : Gain  Gain=1/reserv_str.DriveSys.ScrewLead
  mm2inch_Output(inch/min) : Gain  Gain=1/25.4
  rev/min : Outport
  wires:
  Rev/inch_Output(rev/min)/1 -> Gear_Input(rev/min)/1
  1/CrossArea_Output(mm/min)/1 -> mm2inch_Output(inch/min)/1
  unit/s/1 -> Gain/1
  mm2inch_Output(inch/min)/1 -> Rev/inch_Output(rev/min)/1
  Gain3/1 -> 1/CrossArea_Output(mm/min)/1  "mm^3/min"
  Gain/1 -> Gain3/1
  Gear_Input(rev/min)/1 -> rev/min/1

== stateflow chart InsulinPumpModelV7_ParFor/Subsystem/BolusChart ==
  state Off
  state NormalBolusMode
    state UnitRemainLow
    state NumCycFinished
    state Deliver
      entry: StrokeMag = MagB/StrokeTimeB;
    state Active
      entry: i = int8(0);
    state Pause
      entry: StrokeMag = single(0);
    state Inactive
      entry:StrokeMag = single(0);
    UnitRemainLow -> (junction 108)
    (junction 108) -> NormalBolusMode.Inactive
    (junction 27) -> UnitRemainLow [order 2] : [UnitRemain<LowLim+MagB]
    NumCycFinished -> (junction 41)
    (junction 41) -> NormalBolusMode.Inactive
    (junction 29) -> NumCycFinished [order 1] : [i>=NumCyc]
    (default) -> NormalBolusMode.Inactive
    Deliver -> (junction 104) : after(StrokeTimeB,sec)
    (junction 104) -> (junction 29) : {i = i + 1;}
    (junction 29) -> (junction 27) [order 2]
    (junction 27) -> Pause [order 1] : [UnitRemain>LowLim+MagB]
    NormalBolusMode.Inactive -> (junction 100) : [UnitRemain>LowLim+MagB]
    (junction 100) -> NormalBolusMode.Active : [DeliveryActive == true]
    NormalBolusMode.Active -> Deliver [order 1] : [i<NumCyc]
    Pause -> Deliver : after(PauseTime,sec)
    NormalBolusMode.Active -> NormalBolusMode.Inactive [order 2] : [UnitRemain<LowLim+MagB]
  state Armed
  state QuickBolusMode
    state Deliver1
      entry: StrokeMag = MagQB (1)/StrokeTimeQB(1);
    state Pause1
      entry: StrokeMag = single(0);
    state Inactive
      entry:StrokeMag = single(0);
    state Active
      entry: i = int8(0);
    state Deliver2
      entry: StrokeMag = MagQB(2)/StrokeTimeQB(2);
    state Pause2
      entry: StrokeMag = single(0);
    state Deliver3
      entry: StrokeMag = MagQB(3)/StrokeTimeQB(3);
    state Pause3
      entry: StrokeMag = single(0);
    state Deliver4
      entry: StrokeMag = MagQB(4)/StrokeTimeQB(4);
    state Pause4
      entry: StrokeMag = single(0);
    (junction 92) -> (junction 90)
    (junction 90) -> Deliver1
    Pause4 -> (junction 92) : after(PauseTime,sec)
    (default) -> QuickBolusMode.Inactive
    QuickBolusMode.Inactive -> (junction 119) : [UnitRemain>LowLim+sum(MagQB)]
    (junction 119) -> QuickBolusMode.Active : [DeliveryActive == true]
    QuickBolusMode.Active -> Deliver1
    Deliver1 -> Pause1 : after(StrokeTimeQB(1),sec)
    Pause1 -> Deliver2 : after(PauseTime,sec)
    (junction 116) -> QuickBolusMode.Inactive
    (junction 85) -> QuickBolusMode.Inactive
    Deliver2 -> Pause2 : after(StrokeTimeQB(2),sec)
    Pause2 -> Deliver3 : after(PauseTime,sec)
    Deliver3 -> Pause3 : after(StrokeTimeQB(3),sec)
    Pause3 -> Deliver4 : after(PauseTime,sec)
    Deliver4 -> (junction 78) : after(StrokeTimeQB(4),sec)
    (junction 78) -> (junction 77) : {i=i+1;}
    (junction 77) -> (junction 112) [order 1] : [i<NumCyc]
    (junction 112) -> Pause4 [order 1] : [UnitRemain>LowLim+sum(MagQB)]
    (junction 77) -> (junction 81) [order 2] : [i>=NumCyc]
    (junction 112) -> (junction 114) [order 2] : [UnitRemain<LowLim+sum(MagQB)]
    (junction 81) -> (junction 85)
    (junction 114) -> (junction 116)
  (default) -> Off
  Off -> Armed : [PowerOn ==true]
  Armed -> Off [order 1] : [PowerOn==false]
  Armed -> NormalBolusMode [order 2] : [DeliveryType ==1]
  NormalBolusMode -> Armed : [DeliveryType~=1]
  Armed -> QuickBolusMode [order 3] : [DeliveryType==2]
  QuickBolusMode -> Armed : [DeliveryType~=2]
  data: PowerOn input boolean [0..1]; DeliveryType input int8 [0..2]; NumCyc input int8 [0..100]; DeliveryActive input boolean [0..1]; MagB input single [0..3]; StrokeMag output [0..15]; i local int8; StrokeTimeB input single [0.2..5]; MagQB input single [0..3]; StrokeTimeQB input single [0.2..5]; PauseTime input single [0..100]; LowLim input single [0..100]; UnitRemain input single [0..201]

== stateflow chart InsulinPumpModelV7_ParFor/Subsystem/BasalChart ==
  state Off
  state On
  state BasalOff
    entry: BasalRate = single(0);
  state BasalOn
    entry:BasalRate = BasalSet;
  (default) -> Off
  Off -> On : [PowerOn ==true]
  On -> Off [order 1] : [PowerOn==false]
  On -> BasalOff [order 2] : [UnitRemain>LowLim]
  BasalOff -> BasalOn [order 2] : [BasalActive==true]
  BasalOn -> BasalOff [order 1] : [BasalActive==false]
  BasalOn -> BasalOff [order 2] : [UnitRemain<LowLim]
  BasalOff -> On [order 1] : [UnitRemain<LowLim]
  data: PowerOn input boolean [0..1]; BasalActive input boolean [0..1]; BasalSet input single [0..2]; LowLim input single [0..100]; UnitRemain input single [0..201]; BasalRate output single [0..2]
